simulink model "TB04_StageB_ClosedLoop"  (R2025a)
settings: Solver=FixedStepDiscrete  StartTime=0  StopTime=TB.t_end  FixedStep=TB.dt  RelTol=1e-3
InitFcn:
  | % 모델과 같은 폴더의 초기화 스크립트를 실행해 P(설계 파라미터)와 TB(시험 조건)를 만든다.
  | run(fullfile(fileparts(get_param(bdroot, 'FileName')), 'TB04_init.m'));
values from neighbouring files (symbols this model uses):
  TB = struct()    [TB04_init.m]
libraries: fl_lib x56, nesl_utility x23
(part 1 of 2)
settings Model: Creator=hj000  LastModifiedBy=hj000
settings DataIOCC: SaveOutput=off  SignalLogging=off  SaveTime=off

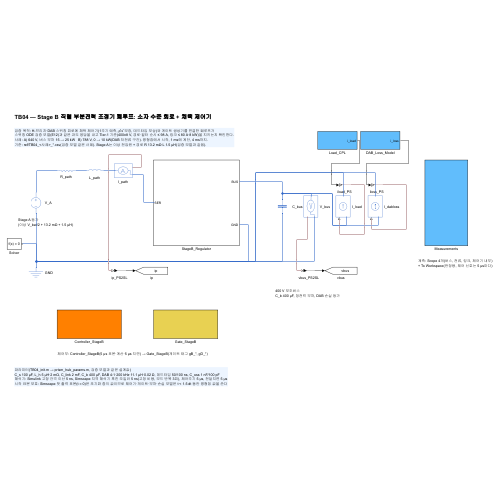
[thumbnail: Simulink's stored preview of the top-level diagram]
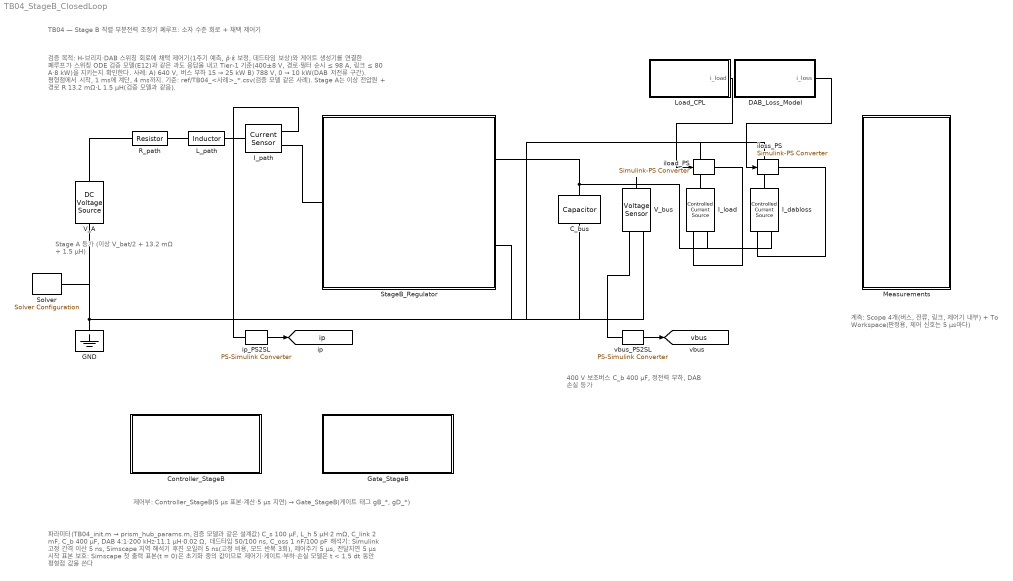
== system TB04_StageB_ClosedLoop ==
  note: TB04 — Stage B 직렬 부분전력 조정기 폐루프: 소자 수준 회로 + 채택 제어기
  note: 검증 목적: H-브리지·DAB 스위칭 회로에 채택 제어기(1주기 예측, ρ̂·ε̂ 보정, 데드타임 보상)와 게이트 생성기를 연결한 폐루프가
      | 스위칭 ODE 검증 모델(E12)과 같은 과도 응답을 내고 Tier-1 기준(400±8 V, 경로·필터 순시 ≤ 98 A, 링크 ≤ 80 A·8 kW)을 지키는지 확인한다.
      | 사례: A) 640 V, 버스 부하 15 → 25 kW   B) 788 V, 0 → 10 kW(DAB 저전류 구간). 평형점에서 시작, 1 ms에 계단, 4 ms까지.
      | 기준: ref/TB04_<사례>_*.csv(검증 모델 같은 사례). Stage A는 이상 전압원 + 경로 R 13.2 mΩ·L 1.5 µH(검증 모델과 같음).
  note: Stage A 등가
      | (이상 V_bat/2 + 13.2 mΩ + 1.5 µH)
  note: 400 V 보조버스
      | C_b 400 µF, 정전력 부하, DAB 손실 등가
  note: 제어부: Controller_StageB(5 µs 표본·계산·5 µs 지연) → Gate_StageB(게이트 태그 gB_*, gD_*)
  note: 계측: Scope 4개(버스, 전류, 링크, 제어기 내부)
      | + To Workspace(판정용, 제어 신호는 5 µs마다)
  note: 파라미터(TB04_init.m → prism_hub_params.m, 검증 모델과 같은 설계값)
      | C_s 100 µF, L_h 5 µH·2 mΩ, C_link 2 mF, C_b 400 µF, DAB 4:1·200 kHz·11.1 µH·0.02 Ω, 데드타임 50/100 ns, C_oss 1 nF/100 pF
      | 해석기: Simulink 고정 간격 이산 5 ns, Simscape 지역 해석기 후진 오일러 5 ns(고정 비용, 모드 반복 3회), 제어주기 5 µs, 전달지연 5 µs
      | 시작 표본 보호: Simscape 첫 출력 표본(t = 0)은 초기화 중의 값이므로 제어기·게이트·부하·손실 모델은 t < 1.5 dt 동안 평형점 값을 쓴다
  C_bus : fl_lib/Electrical/Electrical Elements/Capacitor  c=TB.Cb F  r=1e-6 Ohm  g=0 1/Ohm  i_specify=off  i_priority=None  i=0 A  i_nominal_specify=off  i_nominal_value=1  i_nominal_unit=A  v_specify=off  v_priority=None  v=0 V  v_nominal_specify=off  v_nominal_value=1  v_nominal_unit=V  vc_specify=on  vc_priority=High  vc=TB.vb0 V  vc_nominal_specify=off  vc_nominal_value=1  vc_nominal_unit=V
  Controller_StageB : Subsystem
  DAB_Loss_Model : Subsystem
  GND : fl_lib/Electrical/Electrical Elements/Electrical Reference
  Gate_StageB : Subsystem
  I_dabloss : fl_lib/Electrical/Electrical Sources/Controlled Current Source
  I_load : fl_lib/Electrical/Electrical Sources/Controlled Current Source
  I_path : fl_lib/Electrical/Electrical Sensors/Current Sensor
  L_path : fl_lib/Electrical/Electrical Elements/Inductor  l=TB.Lpath H  r=0 Ohm  g=1e-9 1/Ohm  i_specify=off  i_priority=None  i=0 A  i_nominal_specify=off  i_nominal_value=1  i_nominal_unit=A  v_specify=off  v_priority=None  v=0 V  v_nominal_specify=off  v_nominal_value=1  v_nominal_unit=V  i_L_specify=on  i_L_priority=High  i_L=TB.ip0 A  i_L_nominal_specify=off  i_L_nominal_value=1  i_L_nominal_unit=A
  Load_CPL : Subsystem
  Measurements : Subsystem
  R_path : fl_lib/Electrical/Electrical Elements/Resistor  R=TB.Rpath Ohm  i_specify=off  i_priority=None  i=0 A  i_nominal_specify=off  i_nominal_value=1  i_nominal_unit=A  v_specify=off  v_priority=None  v=0 V  v_nominal_specify=off  v_nominal_value=1  v_nominal_unit=V
  Solver : nesl_utility/Solver Configuration  PhysicalDomain=network_engine_domain  SubClassName=solver  LeftPortType=input  RightPortType=generic  Tones=[]  Harmonics=[]  SimulateNoise=off  Profile=off  UseLocalSampling=off  EnableSwitchedLinearOptims=on  FrequencyDomain=off  UseCCode=off  RelTol=0.001  AbsTol=0.001  MinStep=1e-09  ToWorkspace=off  RevertToSquareIcSolve=off  NumHomotopyIterations=100  PhasorMode=off  PhasorModeNumHarmonics=1  ConsistencySolver=NEWTON_XTOL_AFTER_FTOL  IndexReductionMethod=DerivativeReplacement  DoDC=off  ResidualTolerance=1e-9  ConsistencyTolSource=GLOBAL  ConsistencyAbsTol=0.001  ConsistencyRelTol=0.001  ConsistencyTolFactor=0.001  UseLocalSolver=on  LocalSolverChoice=NE_BACKWARD_EULER_ADVANCER  ResolveIndetEquations=on  FunctionEvalNumThread=1  LocalSolverSampleTime=TB.dt  DoFixedCost=on  MaxNonlinIter=3  MaxModeIter=2  ComputeImpulses=off  ImpulseIterations=2  LinearAlgebra=auto  LinearAlgebraNumThread=0  EquationFormulation=NE_TIME_EF  DelaysMemoryBudget=1024  AutomaticFiltering=on  FilteringTimeConstant=0.001  PartitionStorageMethod=AS_NEEDED  PartitionMemoryBudget=1024  PartitionMethod=ROBUST  MultibodyUseLocalSolver=off  MultibodyLocalSolverChoice=ODE1  MultibodyLocalSolverSampleTime=0.001
  StageB_Regulator : Subsystem
  V_A : fl_lib/Electrical/Electrical Sources/DC Voltage Source  v0=TB.VA V
  V_bus : fl_lib/Electrical/Electrical Sensors/Voltage Sensor
  iload_PS : nesl_utility/Simulink-PS Converter  PhysicalDomain=network_engine_domain  SubClassName=ps_input  LeftPortType=input  RightPortType=output  PseudoPeriodic=off  Frequencies=[]  NoiseDistribution=none  NoiseParameters=[]  Unit=1  AffineConversion=off  FilteringAndDerivatives=provide  SimscapeFilterOrder=1  InputFilterTimeConstant=0.001  UdotUserProvided=0
  iloss_PS : nesl_utility/Simulink-PS Converter  PhysicalDomain=network_engine_domain  SubClassName=ps_input  LeftPortType=input  RightPortType=output  PseudoPeriodic=off  Frequencies=[]  NoiseDistribution=none  NoiseParameters=[]  Unit=1  AffineConversion=off  FilteringAndDerivatives=provide  SimscapeFilterOrder=1  InputFilterTimeConstant=0.001  UdotUserProvided=0
  ip_PS2SL : nesl_utility/PS-Simulink Converter  PhysicalDomain=network_engine_domain  SubClassName=ps_output  LeftPortType=input  RightPortType=output  PseudoPeriodic=off  Frequencies=[]  VectorFormat=inherit  Unit=inherit  AffineConversion=off
  vbus_PS2SL : nesl_utility/PS-Simulink Converter  PhysicalDomain=network_engine_domain  SubClassName=ps_output  LeftPortType=input  RightPortType=output  PseudoPeriodic=off  Frequencies=[]  VectorFormat=inherit  Unit=inherit  AffineConversion=off
  tag scope: ip=global, vbus=global
  wires:
  ip_PS2SL/1 -> [ip]
  vbus_PS2SL/1 -> [vbus]
  Load_CPL/1(i_load) -> iload_PS/1
  DAB_Loss_Model/1(i_loss) -> iloss_PS/1
  connections:
  Solver/RConn1 -- V_A/RConn1 -- StageB_Regulator/RConn2 -- C_bus/RConn1 -- V_bus/RConn2 -- I_load/LConn1 -- GND/LConn1 -- I_dabloss/LConn1
  V_A/LConn1 -- R_path/LConn1
  R_path/RConn1 -- L_path/LConn1
  L_path/RConn1 -- I_path/LConn1
  I_path/RConn2 -- StageB_Regulator/LConn1
  StageB_Regulator/RConn1 -- V_bus/LConn1 -- I_load/RConn2 -- C_bus/LConn1 -- I_dabloss/RConn2
  iload_PS/RConn1 -- I_load/RConn1
  iloss_PS/RConn1 -- I_dabloss/RConn1
  I_path/RConn1 -- ip_PS2SL/LConn1
  V_bus/RConn1 -- vbus_PS2SL/LConn1

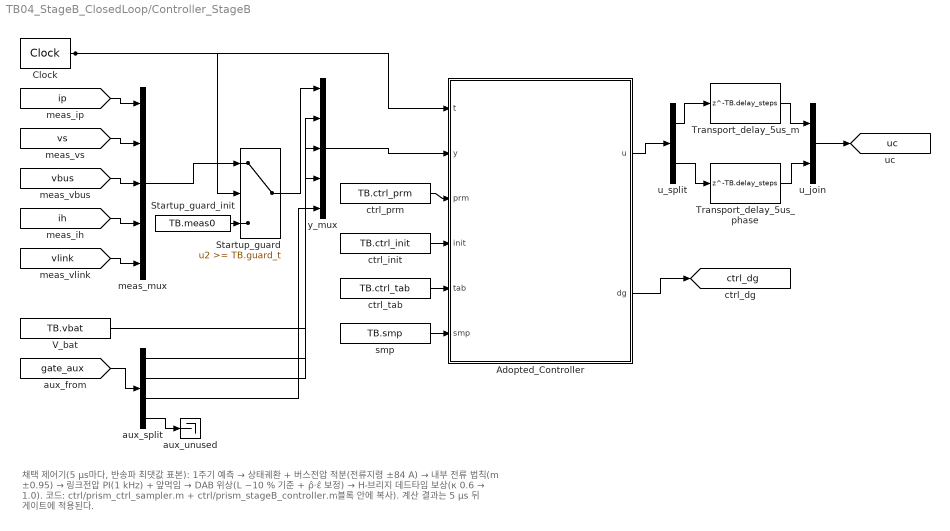
== system TB04_StageB_ClosedLoop/Controller_StageB ==
  note: 채택 제어기(5 µs마다, 반송파 최댓값 표본): 1주기 예측 → 상태궤환 + 버스전압 적분(전류지령 ±84 A) → 내부 전류 법칙(m ±0.95)
      | → 링크전압 PI(1 kHz) + 앞먹임 → DAB 위상(L −10 % 기준 + ρ̂·ε̂ 보정) → H-브리지 데드타임 보상(κ 0.6 → 1.0).
      | 코드: ctrl/prism_ctrl_sampler.m + ctrl/prism_stageB_controller.m(블록 안에 복사). 계산 결과는 5 µs 뒤 게이트에 적용된다.
  Adopted_Controller : MATLAB Function  TreatAsAtomicUnit=on
  Clock : DigitalClock  SampleTime=TB.dt
  Startup_guard : Switch  Threshold=TB.guard_t  SaturateOnIntegerOverflow=off  InputSameDT=off
  Startup_guard_init : Constant  Value=TB.meas0
  Transport_delay_5us_m : Delay  DelayLength=TB.delay_steps  InitialCondition=TB.uc0(1)
  Transport_delay_5us_phase : Delay  DelayLength=TB.delay_steps  InitialCondition=TB.uc0(2)
  V_bat : Constant  Value=TB.vbat
  aux_split : Demux  Outputs=[1 1 1 3]
  aux_unused : Terminator
  ctrl_init : Constant  Value=TB.ctrl_init
  ctrl_prm : Constant  Value=TB.ctrl_prm
  ctrl_tab : Constant  Value=TB.ctrl_tab
  meas_mux : Mux  Inputs=5
  smp : Constant  Value=TB.smp
  u_join : Mux  Inputs=2
  u_split : Demux  Outputs=2
  y_mux : Mux  Inputs=5
  tag scope: ctrl_dg=global, uc=global
  wires:
  [ip] -> meas_mux/1
  [vs] -> meas_mux/2
  [vbus] -> meas_mux/3
  [ih] -> meas_mux/4
  [vlink] -> meas_mux/5
  Startup_guard_init/1 -> Startup_guard/3
  meas_mux/1 -> Startup_guard/1
  Clock/1 -> Startup_guard/2, Adopted_Controller/1(t)
  Startup_guard/1 -> y_mux/1
  V_bat/1 -> y_mux/2
  [gate_aux] -> aux_split/1
  aux_split/1 -> y_mux/3
  aux_split/2 -> y_mux/4
  aux_split/3 -> y_mux/5
  aux_split/4 -> aux_unused/1
  y_mux/1 -> Adopted_Controller/2(y)
  ctrl_prm/1 -> Adopted_Controller/3(prm)
  ctrl_init/1 -> Adopted_Controller/4(init)
  ctrl_tab/1 -> Adopted_Controller/5(tab)
  smp/1 -> Adopted_Controller/6(smp)
  Adopted_Controller/1(u) -> u_split/1
  u_split/1 -> Transport_delay_5us_m/1
  u_split/2 -> Transport_delay_5us_phase/1
  Transport_delay_5us_m/1 -> u_join/1
  Transport_delay_5us_phase/1 -> u_join/2
  u_join/1 -> [uc]
  Adopted_Controller/2(dg) -> [ctrl_dg]

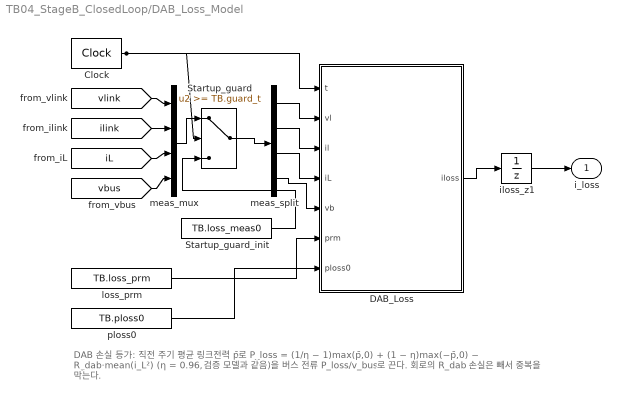
== system TB04_StageB_ClosedLoop/DAB_Loss_Model ==
  note: DAB 손실 등가: 직전 주기 평균 링크전력 p̄로 P_loss = (1/η − 1)max(p̄,0) + (1 − η)max(−p̄,0) − R_dab·mean(i_L²)
      | (η = 0.96, 검증 모델과 같음)을 버스 전류 P_loss/v_bus로 끈다. 회로의 R_dab 손실은 빼서 중복을 막는다.
  Clock : DigitalClock  SampleTime=TB.dt
  DAB_Loss : MATLAB Function  TreatAsAtomicUnit=on
  Startup_guard : Switch  Threshold=TB.guard_t  SaturateOnIntegerOverflow=off  InputSameDT=off
  Startup_guard_init : Constant  Value=TB.loss_meas0
  iloss_z1 : UnitDelay  SampleTime=TB.dt  HasFrameUpgradeWarning=on
  loss_prm : Constant  Value=TB.loss_prm
  meas_mux : Mux
  meas_split : Demux
  ploss0 : Constant  Value=TB.ploss0
  i_loss : Outport
  wires:
  [vlink] -> meas_mux/1
  [ilink] -> meas_mux/2
  [iL] -> meas_mux/3
  [vbus] -> meas_mux/4
  Startup_guard_init/1 -> Startup_guard/3
  meas_mux/1 -> Startup_guard/1
  Clock/1 -> Startup_guard/2, DAB_Loss/1(t)
  Startup_guard/1 -> meas_split/1
  meas_split/1 -> DAB_Loss/2(vl)
  meas_split/2 -> DAB_Loss/3(il)
  meas_split/3 -> DAB_Loss/4(iL)
  meas_split/4 -> DAB_Loss/5(vb)
  loss_prm/1 -> DAB_Loss/6(prm)
  ploss0/1 -> DAB_Loss/7(ploss0)
  DAB_Loss/1(iloss) -> iloss_z1/1
  iloss_z1/1 -> i_loss/1

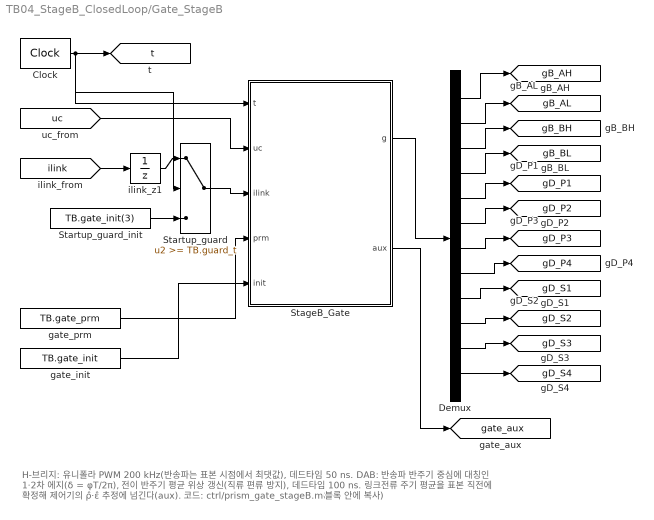
== system TB04_StageB_ClosedLoop/Gate_StageB ==
  note: H-브리지: 유니폴라 PWM 200 kHz(반송파는 표본 시점에서 최댓값), 데드타임 50 ns.
      | DAB: 반송파 반주기 중심에 대칭인 1·2차 에지(δ = φT/2π), 전이 반주기 평균 위상 갱신(직류 편류 방지), 데드타임 100 ns.
      | 링크전류 주기 평균을 표본 직전에 확정해 제어기의 ρ̂·ε̂ 추정에 넘긴다(aux). 코드: ctrl/prism_gate_stageB.m(블록 안에 복사)
  Clock : DigitalClock  SampleTime=TB.dt
  Demux : Demux  Outputs=12
  StageB_Gate : MATLAB Function  TreatAsAtomicUnit=on
  Startup_guard : Switch  Threshold=TB.guard_t  SaturateOnIntegerOverflow=off  InputSameDT=off
  Startup_guard_init : Constant  Value=TB.gate_init(3)
  gate_init : Constant  Value=TB.gate_init
  gate_prm : Constant  Value=TB.gate_prm
  ilink_z1 : UnitDelay  SampleTime=TB.dt  HasFrameUpgradeWarning=on
  tag scope: gB_AH=global, gB_AL=global, gB_BH=global, gB_BL=global, gD_P1=global, gD_P2=global, gD_P3=global, gD_P4=global, gD_S1=global, gD_S2=global, gD_S3=global, gD_S4=global, gate_aux=global, t=global
  wires:
  Startup_guard_init/1 -> Startup_guard/3
  Clock/1 -> [t], StageB_Gate/1(t), Startup_guard/2
  [uc] -> StageB_Gate/2(uc)
  [ilink] -> ilink_z1/1
  ilink_z1/1 -> Startup_guard/1
  Startup_guard/1 -> StageB_Gate/3(ilink)
  gate_prm/1 -> StageB_Gate/4(prm)
  gate_init/1 -> StageB_Gate/5(init)
  StageB_Gate/1(g) -> Demux/1
  Demux/1 -> [gB_AH]
  Demux/2 -> [gB_AL]
  Demux/3 -> [gB_BH]
  Demux/4 -> [gB_BL]
  Demux/5 -> [gD_P1]
  Demux/6 -> [gD_P2]
  Demux/7 -> [gD_P3]
  Demux/8 -> [gD_P4]
  Demux/9 -> [gD_S1]
  Demux/10 -> [gD_S2]
  Demux/11 -> [gD_S3]
  Demux/12 -> [gD_S4]
  StageB_Gate/2(aux) -> [gate_aux]

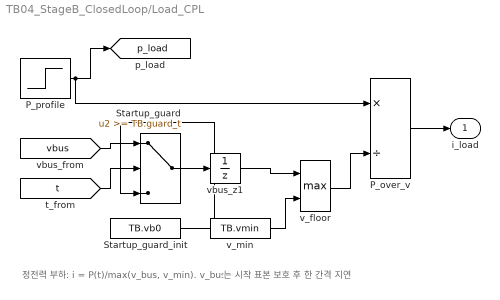
== system TB04_StageB_ClosedLoop/Load_CPL ==
  note: 정전력 부하: i = P(t)/max(v_bus, v_min). v_bus는 시작 표본 보호 후 한 간격 지연
  P_over_v : Product  Inputs=*/
  P_profile : Step  Time=TB.t_step  Before=TB.P0  After=TB.P1  SampleTime=TB.dt
  Startup_guard : Switch  Threshold=TB.guard_t  SaturateOnIntegerOverflow=off  InputSameDT=off
  Startup_guard_init : Constant  Value=TB.vb0
  v_floor : MinMax  Function=max  Inputs=2
  v_min : Constant  Value=TB.vmin
  vbus_z1 : UnitDelay  SampleTime=TB.dt  HasFrameUpgradeWarning=on
  i_load : Outport
  tag scope: p_load=global
  wires:
  Startup_guard_init/1 -> Startup_guard/3
  P_profile/1 -> [p_load], P_over_v/1
  [vbus] -> Startup_guard/1
  [t] -> Startup_guard/2
  Startup_guard/1 -> vbus_z1/1
  vbus_z1/1 -> v_floor/1
  v_min/1 -> v_floor/2
  v_floor/1 -> P_over_v/2
  P_over_v/1 -> i_load/1

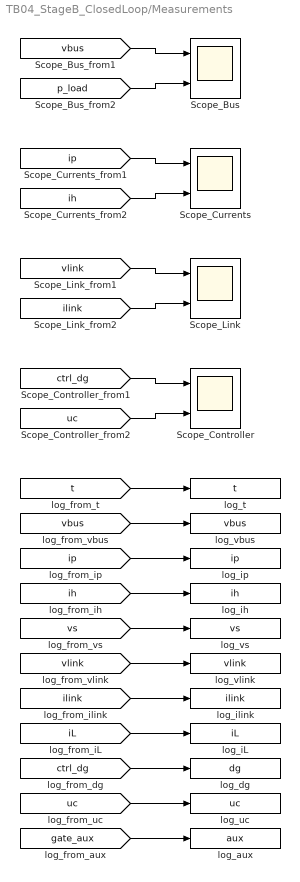
== system TB04_StageB_ClosedLoop/Measurements ==
  Scope_Bus : Scope  NumInputPorts=2
      settings: Title=Scope Bus
  Scope_Controller : Scope  NumInputPorts=2
      settings: Title=Scope Controller
  Scope_Currents : Scope  NumInputPorts=2
      settings: Title=Scope Currents
  Scope_Link : Scope  NumInputPorts=2
      settings: Title=Scope Link
  log_aux : ToWorkspace  VariableName=aux  SampleTime=-1
      settings: Decimation=TB.Np
  log_dg : ToWorkspace  VariableName=dg  SampleTime=-1
      settings: Decimation=TB.Np
  log_iL : ToWorkspace  VariableName=iL  SampleTime=-1
  log_ih : ToWorkspace  VariableName=ih  SampleTime=-1
  log_ilink : ToWorkspace  VariableName=ilink  SampleTime=-1
  log_ip : ToWorkspace  VariableName=ip  SampleTime=-1
  log_t : ToWorkspace  VariableName=t  SampleTime=-1
  log_uc : ToWorkspace  VariableName=uc  SampleTime=-1
      settings: Decimation=TB.Np
  log_vbus : ToWorkspace  VariableName=vbus  SampleTime=-1
  log_vlink : ToWorkspace  VariableName=vlink  SampleTime=-1
  log_vs : ToWorkspace  VariableName=vs  SampleTime=-1
  wires:
  [vbus] -> Scope_Bus/1
  [p_load] -> Scope_Bus/2
  [ip] -> Scope_Currents/1
  [ih] -> Scope_Currents/2
  [vlink] -> Scope_Link/1
  [ilink] -> Scope_Link/2
  [ctrl_dg] -> Scope_Controller/1
  [uc] -> Scope_Controller/2
  [t] -> log_t/1
  [vbus] -> log_vbus/1
  [ip] -> log_ip/1
  [ih] -> log_ih/1
  [vs] -> log_vs/1
  [vlink] -> log_vlink/1
  [ilink] -> log_ilink/1
  [iL] -> log_iL/1
  [ctrl_dg] -> log_dg/1
  [uc] -> log_uc/1
  [gate_aux] -> log_aux/1

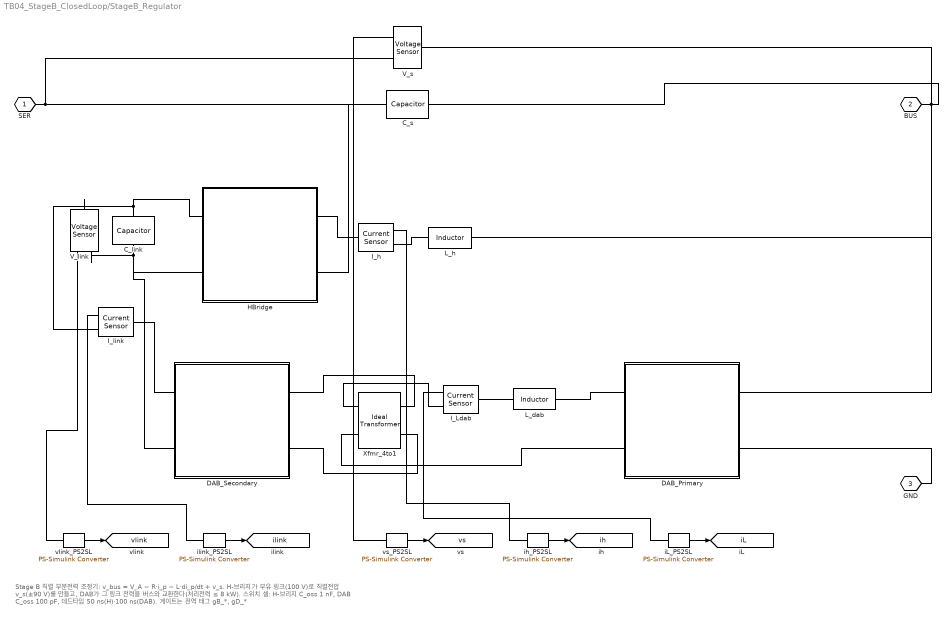
== system TB04_StageB_ClosedLoop/StageB_Regulator ==
  note: Stage B 직렬 부분전력 조정기: v_bus = V_A − R·i_p − L·di_p/dt + v_s.
      | H-브리지가 부유 링크(100 V)로 직렬전압 v_s(±90 V)를 만들고, DAB가 그 링크 전력을 버스와 교환한다(처리전력 ≤ 8 kW).
      | 스위치 셀: H-브리지 C_oss 1 nF, DAB C_oss 100 pF, 데드타임 50 ns(H)·100 ns(DAB). 게이트는 전역 태그 gB_*, gD_*
  C_link : fl_lib/Electrical/Electrical Elements/Capacitor  c=TB.B.Clink F  r=1e-6 Ohm  g=0 1/Ohm  i_specify=off  i_priority=None  i=0 A  i_nominal_specify=off  i_nominal_value=1  i_nominal_unit=A  v_specify=off  v_priority=None  v=0 V  v_nominal_specify=off  v_nominal_value=1  v_nominal_unit=V  vc_specify=on  vc_priority=High  vc=TB.vl0 V  vc_nominal_specify=off  vc_nominal_value=1  vc_nominal_unit=V
  C_s : fl_lib/Electrical/Electrical Elements/Capacitor  c=TB.B.Cs F  r=1e-6 Ohm  g=0 1/Ohm  i_specify=off  i_priority=None  i=0 A  i_nominal_specify=off  i_nominal_value=1  i_nominal_unit=A  v_specify=off  v_priority=None  v=0 V  v_nominal_specify=off  v_nominal_value=1  v_nominal_unit=V  vc_specify=on  vc_priority=High  vc=TB.vs0 V  vc_nominal_specify=off  vc_nominal_value=1  vc_nominal_unit=V
  DAB_Primary : Subsystem
  DAB_Secondary : Subsystem
  HBridge : Subsystem
  I_Ldab : fl_lib/Electrical/Electrical Sensors/Current Sensor
  I_h : fl_lib/Electrical/Electrical Sensors/Current Sensor
  I_link : fl_lib/Electrical/Electrical Sensors/Current Sensor
  L_dab : fl_lib/Electrical/Electrical Elements/Inductor  l=TB.B.Ldab H  r=TB.B.Rdab Ohm  g=1e-9 1/Ohm  i_specify=off  i_priority=None  i=0 A  i_nominal_specify=off  i_nominal_value=1  i_nominal_unit=A  v_specify=off  v_priority=None  v=0 V  v_nominal_specify=off  v_nominal_value=1  v_nominal_unit=V  i_L_specify=on  i_L_priority=High  i_L=0 A  i_L_nominal_specify=off  i_L_nominal_value=1  i_L_nominal_unit=A
  L_h : fl_lib/Electrical/Electrical Elements/Inductor  l=TB.B.Lh H  r=TB.B.Rh Ohm  g=1e-9 1/Ohm  i_specify=off  i_priority=None  i=0 A  i_nominal_specify=off  i_nominal_value=1  i_nominal_unit=A  v_specify=off  v_priority=None  v=0 V  v_nominal_specify=off  v_nominal_value=1  v_nominal_unit=V  i_L_specify=on  i_L_priority=High  i_L=TB.ih0 A  i_L_nominal_specify=off  i_L_nominal_value=1  i_L_nominal_unit=A
  V_link : fl_lib/Electrical/Electrical Sensors/Voltage Sensor
  V_s : fl_lib/Electrical/Electrical Sensors/Voltage Sensor
  Xfmr_4to1 : fl_lib/Electrical/Electrical Elements/Ideal Transformer  n=TB.B.n  i1_specify=off  i1_priority=None  i1=0 A  i1_nominal_specify=off  i1_nominal_value=1  i1_nominal_unit=A  v1_specify=off  v1_priority=None  v1=0 V  v1_nominal_specify=off  v1_nominal_value=1  v1_nominal_unit=V  i2_specify=off  i2_priority=None  i2=0 A  i2_nominal_specify=off  i2_nominal_value=1  i2_nominal_unit=A  v2_specify=off  v2_priority=None  v2=0 V  v2_nominal_specify=off  v2_nominal_value=1  v2_nominal_unit=V
  iL_PS2SL : nesl_utility/PS-Simulink Converter  PhysicalDomain=network_engine_domain  SubClassName=ps_output  LeftPortType=input  RightPortType=output  PseudoPeriodic=off  Frequencies=[]  VectorFormat=inherit  Unit=inherit  AffineConversion=off
  ih_PS2SL : nesl_utility/PS-Simulink Converter  PhysicalDomain=network_engine_domain  SubClassName=ps_output  LeftPortType=input  RightPortType=output  PseudoPeriodic=off  Frequencies=[]  VectorFormat=inherit  Unit=inherit  AffineConversion=off
  ilink_PS2SL : nesl_utility/PS-Simulink Converter  PhysicalDomain=network_engine_domain  SubClassName=ps_output  LeftPortType=input  RightPortType=output  PseudoPeriodic=off  Frequencies=[]  VectorFormat=inherit  Unit=inherit  AffineConversion=off
  vlink_PS2SL : nesl_utility/PS-Simulink Converter  PhysicalDomain=network_engine_domain  SubClassName=ps_output  LeftPortType=input  RightPortType=output  PseudoPeriodic=off  Frequencies=[]  VectorFormat=inherit  Unit=inherit  AffineConversion=off
  vs_PS2SL : nesl_utility/PS-Simulink Converter  PhysicalDomain=network_engine_domain  SubClassName=ps_output  LeftPortType=input  RightPortType=output  PseudoPeriodic=off  Frequencies=[]  VectorFormat=inherit  Unit=inherit  AffineConversion=off
  SER : PMIOPort  Side=Left
  BUS : PMIOPort  Port=2  Side=Right
  GND : PMIOPort  Port=3  Side=Right
  tag scope: iL=global, ih=global, ilink=global, vlink=global, vs=global
  wires:
  vs_PS2SL/1 -> [vs]
  ih_PS2SL/1 -> [ih]
  vlink_PS2SL/1 -> [vlink]
  ilink_PS2SL/1 -> [ilink]
  iL_PS2SL/1 -> [iL]
  connections:
  C_s/RConn1 -- V_s/RConn2 -- SER/RConn1 -- HBridge/RConn2
  C_s/LConn1 -- V_s/LConn1 -- L_h/RConn1 -- BUS/RConn1 -- DAB_Primary/LConn1
  HBridge/RConn1 -- I_h/LConn1
  I_h/RConn2 -- L_h/LConn1
  HBridge/LConn1 -- C_link/LConn1 -- V_link/LConn1 -- I_link/RConn2
  HBridge/LConn2 -- C_link/RConn1 -- V_link/RConn2 -- DAB_Secondary/LConn2
  DAB_Secondary/LConn1 -- I_link/LConn1
  DAB_Secondary/RConn1 -- Xfmr_4to1/RConn1
  DAB_Secondary/RConn2 -- Xfmr_4to1/RConn2
  DAB_Primary/RConn1 -- L_dab/LConn1
  L_dab/RConn1 -- I_Ldab/LConn1
  I_Ldab/RConn2 -- Xfmr_4to1/LConn1
  Xfmr_4to1/LConn2 -- DAB_Primary/RConn2
  DAB_Primary/LConn2 -- GND/RConn1
  V_s/RConn1 -- vs_PS2SL/LConn1
  I_h/RConn1 -- ih_PS2SL/LConn1
  V_link/RConn1 -- vlink_PS2SL/LConn1
  I_link/RConn1 -- ilink_PS2SL/LConn1
  I_Ldab/RConn1 -- iL_PS2SL/LConn1

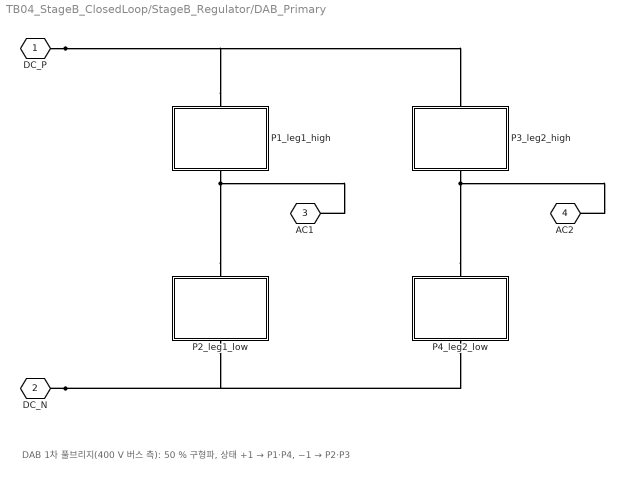
== system TB04_StageB_ClosedLoop/StageB_Regulator/DAB_Primary ==
  note: DAB 1차 풀브리지(400 V 버스 측): 50 % 구형파, 상태 +1 → P1·P4, −1 → P2·P3
  P1_leg1_high : Subsystem  mask(PRISM-Hub switch cell){Ron=TB.B.Ron, Goff=TB.B.Goff, Vf=TB.B.Vf, Rd=TB.B.Rd, Goffd=TB.B.Goffd, Coss=TB.B.Coss_d}
      mask prompts: Ron "도통 저항 R_on [Ohm]"; Goff "차단 컨덕턴스 G_off [S]"; Vf "다이오드 순방향 전압 Vf [V]"; Rd "다이오드 도통 저항 R_d [Ohm]"; Goffd "다이오드 차단 컨덕턴스 [S]"; Coss "출력용량 C_oss [F]"
      mask help: 전력 반도체 스위치 셀 P1_leg1_high. 게이트 태그 gD_P1.
      settings: AttributesFormatString=gate: gD_P1
      mask Display:
      | plot([0.50 0.50 ],[0.95 0.65 ],[0.50 0.74 ],[0.65 0.35 ],[0.50 0.50 ],[0.35 0.05 ]);
      | plot([0.50 0.20 0.20 ],[0.80 0.80 0.58 ],[0.20 0.20 0.50 ],[0.42 0.20 0.20 ]);
      | plot([0.20 0.10 0.30 0.20 ],[0.58 0.42 0.42 0.58 ],[0.10 0.30 ],[0.58 0.58 ]);
      | port_label('LConn',1,'D');
      | port_label('RConn',1,'S');
  P2_leg1_low : Subsystem  mask(PRISM-Hub switch cell){Ron=TB.B.Ron, Goff=TB.B.Goff, Vf=TB.B.Vf, Rd=TB.B.Rd, Goffd=TB.B.Goffd, Coss=TB.B.Coss_d}
      mask prompts: Ron "도통 저항 R_on [Ohm]"; Goff "차단 컨덕턴스 G_off [S]"; Vf "다이오드 순방향 전압 Vf [V]"; Rd "다이오드 도통 저항 R_d [Ohm]"; Goffd "다이오드 차단 컨덕턴스 [S]"; Coss "출력용량 C_oss [F]"
      mask help: 전력 반도체 스위치 셀 P2_leg1_low. 게이트 태그 gD_P2.
      settings: AttributesFormatString=gate: gD_P2
      mask Display:
      | plot([0.50 0.50 ],[0.95 0.65 ],[0.50 0.74 ],[0.65 0.35 ],[0.50 0.50 ],[0.35 0.05 ]);
      | plot([0.50 0.20 0.20 ],[0.80 0.80 0.58 ],[0.20 0.20 0.50 ],[0.42 0.20 0.20 ]);
      | plot([0.20 0.10 0.30 0.20 ],[0.58 0.42 0.42 0.58 ],[0.10 0.30 ],[0.58 0.58 ]);
      | port_label('LConn',1,'D');
      | port_label('RConn',1,'S');
  P3_leg2_high : Subsystem  mask(PRISM-Hub switch cell){Ron=TB.B.Ron, Goff=TB.B.Goff, Vf=TB.B.Vf, Rd=TB.B.Rd, Goffd=TB.B.Goffd, Coss=TB.B.Coss_d}
      mask prompts: Ron "도통 저항 R_on [Ohm]"; Goff "차단 컨덕턴스 G_off [S]"; Vf "다이오드 순방향 전압 Vf [V]"; Rd "다이오드 도통 저항 R_d [Ohm]"; Goffd "다이오드 차단 컨덕턴스 [S]"; Coss "출력용량 C_oss [F]"
      mask help: 전력 반도체 스위치 셀 P3_leg2_high. 게이트 태그 gD_P3.
      settings: AttributesFormatString=gate: gD_P3
      mask Display:
      | plot([0.50 0.50 ],[0.95 0.65 ],[0.50 0.74 ],[0.65 0.35 ],[0.50 0.50 ],[0.35 0.05 ]);
      | plot([0.50 0.20 0.20 ],[0.80 0.80 0.58 ],[0.20 0.20 0.50 ],[0.42 0.20 0.20 ]);
      | plot([0.20 0.10 0.30 0.20 ],[0.58 0.42 0.42 0.58 ],[0.10 0.30 ],[0.58 0.58 ]);
      | port_label('LConn',1,'D');
      | port_label('RConn',1,'S');
  P4_leg2_low : Subsystem  mask(PRISM-Hub switch cell){Ron=TB.B.Ron, Goff=TB.B.Goff, Vf=TB.B.Vf, Rd=TB.B.Rd, Goffd=TB.B.Goffd, Coss=TB.B.Coss_d}
      mask prompts: Ron "도통 저항 R_on [Ohm]"; Goff "차단 컨덕턴스 G_off [S]"; Vf "다이오드 순방향 전압 Vf [V]"; Rd "다이오드 도통 저항 R_d [Ohm]"; Goffd "다이오드 차단 컨덕턴스 [S]"; Coss "출력용량 C_oss [F]"
      mask help: 전력 반도체 스위치 셀 P4_leg2_low. 게이트 태그 gD_P4.
      settings: AttributesFormatString=gate: gD_P4
      mask Display:
      | plot([0.50 0.50 ],[0.95 0.65 ],[0.50 0.74 ],[0.65 0.35 ],[0.50 0.50 ],[0.35 0.05 ]);
      | plot([0.50 0.20 0.20 ],[0.80 0.80 0.58 ],[0.20 0.20 0.50 ],[0.42 0.20 0.20 ]);
      | plot([0.20 0.10 0.30 0.20 ],[0.58 0.42 0.42 0.58 ],[0.10 0.30 ],[0.58 0.58 ]);
      | port_label('LConn',1,'D');
      | port_label('RConn',1,'S');
  DC_P : PMIOPort  Side=Left
  DC_N : PMIOPort  Port=2  Side=Left
  AC1 : PMIOPort  Port=3  Side=Right
  AC2 : PMIOPort  Port=4  Side=Right
  connections:
  P1_leg1_high/LConn1 -- DC_P/RConn1 -- P3_leg2_high/LConn1
  P2_leg1_low/LConn1 -- P1_leg1_high/RConn1 -- AC1/RConn1
  P4_leg2_low/LConn1 -- P3_leg2_high/RConn1 -- AC2/RConn1
  DC_N/RConn1 -- P2_leg1_low/RConn1 -- P4_leg2_low/RConn1

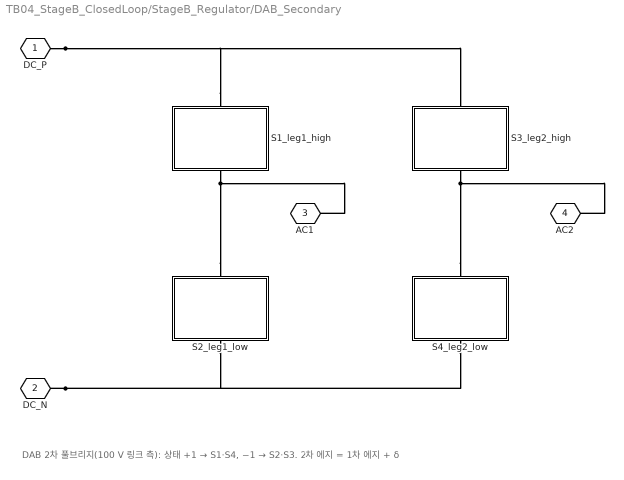
== system TB04_StageB_ClosedLoop/StageB_Regulator/DAB_Secondary ==
  note: DAB 2차 풀브리지(100 V 링크 측): 상태 +1 → S1·S4, −1 → S2·S3. 2차 에지 = 1차 에지 + δ
  S1_leg1_high : Subsystem  mask(PRISM-Hub switch cell){Ron=TB.B.Ron, Goff=TB.B.Goff, Vf=TB.B.Vf, Rd=TB.B.Rd, Goffd=TB.B.Goffd, Coss=TB.B.Coss_d}
      mask prompts: Ron "도통 저항 R_on [Ohm]"; Goff "차단 컨덕턴스 G_off [S]"; Vf "다이오드 순방향 전압 Vf [V]"; Rd "다이오드 도통 저항 R_d [Ohm]"; Goffd "다이오드 차단 컨덕턴스 [S]"; Coss "출력용량 C_oss [F]"
      mask help: 전력 반도체 스위치 셀 S1_leg1_high. 게이트 태그 gD_S1.
      settings: AttributesFormatString=gate: gD_S1
      mask Display:
      | plot([0.50 0.50 ],[0.95 0.65 ],[0.50 0.74 ],[0.65 0.35 ],[0.50 0.50 ],[0.35 0.05 ]);
      | plot([0.50 0.20 0.20 ],[0.80 0.80 0.58 ],[0.20 0.20 0.50 ],[0.42 0.20 0.20 ]);
      | plot([0.20 0.10 0.30 0.20 ],[0.58 0.42 0.42 0.58 ],[0.10 0.30 ],[0.58 0.58 ]);
      | port_label('LConn',1,'D');
      | port_label('RConn',1,'S');
  S2_leg1_low : Subsystem  mask(PRISM-Hub switch cell){Ron=TB.B.Ron, Goff=TB.B.Goff, Vf=TB.B.Vf, Rd=TB.B.Rd, Goffd=TB.B.Goffd, Coss=TB.B.Coss_d}
      mask prompts: Ron "도통 저항 R_on [Ohm]"; Goff "차단 컨덕턴스 G_off [S]"; Vf "다이오드 순방향 전압 Vf [V]"; Rd "다이오드 도통 저항 R_d [Ohm]"; Goffd "다이오드 차단 컨덕턴스 [S]"; Coss "출력용량 C_oss [F]"
      mask help: 전력 반도체 스위치 셀 S2_leg1_low. 게이트 태그 gD_S2.
      settings: AttributesFormatString=gate: gD_S2
      mask Display:
      | plot([0.50 0.50 ],[0.95 0.65 ],[0.50 0.74 ],[0.65 0.35 ],[0.50 0.50 ],[0.35 0.05 ]);
      | plot([0.50 0.20 0.20 ],[0.80 0.80 0.58 ],[0.20 0.20 0.50 ],[0.42 0.20 0.20 ]);
      | plot([0.20 0.10 0.30 0.20 ],[0.58 0.42 0.42 0.58 ],[0.10 0.30 ],[0.58 0.58 ]);
      | port_label('LConn',1,'D');
      | port_label('RConn',1,'S');
  S3_leg2_high : Subsystem  mask(PRISM-Hub switch cell){Ron=TB.B.Ron, Goff=TB.B.Goff, Vf=TB.B.Vf, Rd=TB.B.Rd, Goffd=TB.B.Goffd, Coss=TB.B.Coss_d}
      mask prompts: Ron "도통 저항 R_on [Ohm]"; Goff "차단 컨덕턴스 G_off [S]"; Vf "다이오드 순방향 전압 Vf [V]"; Rd "다이오드 도통 저항 R_d [Ohm]"; Goffd "다이오드 차단 컨덕턴스 [S]"; Coss "출력용량 C_oss [F]"
      mask help: 전력 반도체 스위치 셀 S3_leg2_high. 게이트 태그 gD_S3.
      settings: AttributesFormatString=gate: gD_S3
      mask Display:
      | plot([0.50 0.50 ],[0.95 0.65 ],[0.50 0.74 ],[0.65 0.35 ],[0.50 0.50 ],[0.35 0.05 ]);
      | plot([0.50 0.20 0.20 ],[0.80 0.80 0.58 ],[0.20 0.20 0.50 ],[0.42 0.20 0.20 ]);
      | plot([0.20 0.10 0.30 0.20 ],[0.58 0.42 0.42 0.58 ],[0.10 0.30 ],[0.58 0.58 ]);
      | port_label('LConn',1,'D');
      | port_label('RConn',1,'S');
  S4_leg2_low : Subsystem  mask(PRISM-Hub switch cell){Ron=TB.B.Ron, Goff=TB.B.Goff, Vf=TB.B.Vf, Rd=TB.B.Rd, Goffd=TB.B.Goffd, Coss=TB.B.Coss_d}
      mask prompts: Ron "도통 저항 R_on [Ohm]"; Goff "차단 컨덕턴스 G_off [S]"; Vf "다이오드 순방향 전압 Vf [V]"; Rd "다이오드 도통 저항 R_d [Ohm]"; Goffd "다이오드 차단 컨덕턴스 [S]"; Coss "출력용량 C_oss [F]"
      mask help: 전력 반도체 스위치 셀 S4_leg2_low. 게이트 태그 gD_S4.
      settings: AttributesFormatString=gate: gD_S4
      mask Display:
      | plot([0.50 0.50 ],[0.95 0.65 ],[0.50 0.74 ],[0.65 0.35 ],[0.50 0.50 ],[0.35 0.05 ]);
      | plot([0.50 0.20 0.20 ],[0.80 0.80 0.58 ],[0.20 0.20 0.50 ],[0.42 0.20 0.20 ]);
      | plot([0.20 0.10 0.30 0.20 ],[0.58 0.42 0.42 0.58 ],[0.10 0.30 ],[0.58 0.58 ]);
      | port_label('LConn',1,'D');
      | port_label('RConn',1,'S');
  DC_P : PMIOPort  Side=Left
  DC_N : PMIOPort  Port=2  Side=Left
  AC1 : PMIOPort  Port=3  Side=Right
  AC2 : PMIOPort  Port=4  Side=Right
  connections:
  S1_leg1_high/LConn1 -- DC_P/RConn1 -- S3_leg2_high/LConn1
  S2_leg1_low/LConn1 -- S1_leg1_high/RConn1 -- AC1/RConn1
  S4_leg2_low/LConn1 -- S3_leg2_high/RConn1 -- AC2/RConn1
  DC_N/RConn1 -- S2_leg1_low/RConn1 -- S4_leg2_low/RConn1

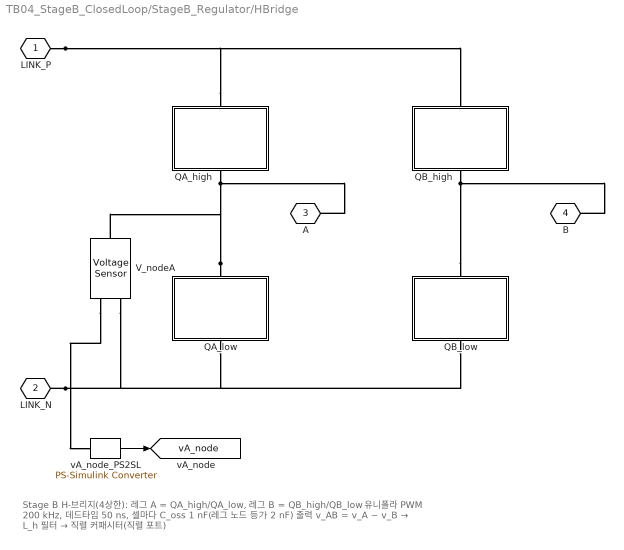
== system TB04_StageB_ClosedLoop/StageB_Regulator/HBridge ==
  note: Stage B H-브리지(4상한): 레그 A = QA_high/QA_low, 레그 B = QB_high/QB_low
      | 유니폴라 PWM 200 kHz, 데드타임 50 ns, 셀마다 C_oss 1 nF(레그 노드 등가 2 nF)
      | 출력 v_AB = v_A − v_B → L_h 필터 → 직렬 커패시터(직렬 포트)
  QA_high : Subsystem  mask(PRISM-Hub switch cell){Ron=TB.B.Ron, Goff=TB.B.Goff, Vf=TB.B.Vf, Rd=TB.B.Rd, Goffd=TB.B.Goffd, Coss=TB.B.Coss_h}
      mask prompts: Ron "도통 저항 R_on [Ohm]"; Goff "차단 컨덕턴스 G_off [S]"; Vf "다이오드 순방향 전압 Vf [V]"; Rd "다이오드 도통 저항 R_d [Ohm]"; Goffd "다이오드 차단 컨덕턴스 [S]"; Coss "출력용량 C_oss [F]"
      mask help: 전력 반도체 스위치 셀 QA_H. 게이트 태그 gB_AH.
      settings: AttributesFormatString=gate: gB_AH
      mask Display:
      | plot([0.50 0.50 ],[0.95 0.65 ],[0.50 0.74 ],[0.65 0.35 ],[0.50 0.50 ],[0.35 0.05 ]);
      | plot([0.50 0.20 0.20 ],[0.80 0.80 0.58 ],[0.20 0.20 0.50 ],[0.42 0.20 0.20 ]);
      | plot([0.20 0.10 0.30 0.20 ],[0.58 0.42 0.42 0.58 ],[0.10 0.30 ],[0.58 0.58 ]);
      | port_label('LConn',1,'D');
      | port_label('RConn',1,'S');
  QA_low : Subsystem  mask(PRISM-Hub switch cell){Ron=TB.B.Ron, Goff=TB.B.Goff, Vf=TB.B.Vf, Rd=TB.B.Rd, Goffd=TB.B.Goffd, Coss=TB.B.Coss_h}
      mask prompts: Ron "도통 저항 R_on [Ohm]"; Goff "차단 컨덕턴스 G_off [S]"; Vf "다이오드 순방향 전압 Vf [V]"; Rd "다이오드 도통 저항 R_d [Ohm]"; Goffd "다이오드 차단 컨덕턴스 [S]"; Coss "출력용량 C_oss [F]"
      mask help: 전력 반도체 스위치 셀 QA_L. 게이트 태그 gB_AL.
      settings: AttributesFormatString=gate: gB_AL
      mask Display:
      | plot([0.50 0.50 ],[0.95 0.65 ],[0.50 0.74 ],[0.65 0.35 ],[0.50 0.50 ],[0.35 0.05 ]);
      | plot([0.50 0.20 0.20 ],[0.80 0.80 0.58 ],[0.20 0.20 0.50 ],[0.42 0.20 0.20 ]);
      | plot([0.20 0.10 0.30 0.20 ],[0.58 0.42 0.42 0.58 ],[0.10 0.30 ],[0.58 0.58 ]);
      | port_label('LConn',1,'D');
      | port_label('RConn',1,'S');
  QB_high : Subsystem  mask(PRISM-Hub switch cell){Ron=TB.B.Ron, Goff=TB.B.Goff, Vf=TB.B.Vf, Rd=TB.B.Rd, Goffd=TB.B.Goffd, Coss=TB.B.Coss_h}
      mask prompts: Ron "도통 저항 R_on [Ohm]"; Goff "차단 컨덕턴스 G_off [S]"; Vf "다이오드 순방향 전압 Vf [V]"; Rd "다이오드 도통 저항 R_d [Ohm]"; Goffd "다이오드 차단 컨덕턴스 [S]"; Coss "출력용량 C_oss [F]"
      mask help: 전력 반도체 스위치 셀 QB_H. 게이트 태그 gB_BH.
      settings: AttributesFormatString=gate: gB_BH
      mask Display:
      | plot([0.50 0.50 ],[0.95 0.65 ],[0.50 0.74 ],[0.65 0.35 ],[0.50 0.50 ],[0.35 0.05 ]);
      | plot([0.50 0.20 0.20 ],[0.80 0.80 0.58 ],[0.20 0.20 0.50 ],[0.42 0.20 0.20 ]);
      | plot([0.20 0.10 0.30 0.20 ],[0.58 0.42 0.42 0.58 ],[0.10 0.30 ],[0.58 0.58 ]);
      | port_label('LConn',1,'D');
      | port_label('RConn',1,'S');
  QB_low : Subsystem  mask(PRISM-Hub switch cell){Ron=TB.B.Ron, Goff=TB.B.Goff, Vf=TB.B.Vf, Rd=TB.B.Rd, Goffd=TB.B.Goffd, Coss=TB.B.Coss_h}
      mask prompts: Ron "도통 저항 R_on [Ohm]"; Goff "차단 컨덕턴스 G_off [S]"; Vf "다이오드 순방향 전압 Vf [V]"; Rd "다이오드 도통 저항 R_d [Ohm]"; Goffd "다이오드 차단 컨덕턴스 [S]"; Coss "출력용량 C_oss [F]"
      mask help: 전력 반도체 스위치 셀 QB_L. 게이트 태그 gB_BL.
      settings: AttributesFormatString=gate: gB_BL
      mask Display:
      | plot([0.50 0.50 ],[0.95 0.65 ],[0.50 0.74 ],[0.65 0.35 ],[0.50 0.50 ],[0.35 0.05 ]);
      | plot([0.50 0.20 0.20 ],[0.80 0.80 0.58 ],[0.20 0.20 0.50 ],[0.42 0.20 0.20 ]);
      | plot([0.20 0.10 0.30 0.20 ],[0.58 0.42 0.42 0.58 ],[0.10 0.30 ],[0.58 0.58 ]);
      | port_label('LConn',1,'D');
      | port_label('RConn',1,'S');
  V_nodeA : fl_lib/Electrical/Electrical Sensors/Voltage Sensor
  vA_node_PS2SL : nesl_utility/PS-Simulink Converter  PhysicalDomain=network_engine_domain  SubClassName=ps_output  LeftPortType=input  RightPortType=output  PseudoPeriodic=off  Frequencies=[]  VectorFormat=inherit  Unit=inherit  AffineConversion=off
  LINK_P : PMIOPort  Side=Left
  LINK_N : PMIOPort  Port=2  Side=Left
  A : PMIOPort  Port=3  Side=Right
  B : PMIOPort  Port=4  Side=Right
  tag scope: vA_node=global
  wires:
  vA_node_PS2SL/1 -> [vA_node]
  connections:
  QA_high/LConn1 -- LINK_P/RConn1 -- QB_high/LConn1
  QA_high/RConn1 -- A/RConn1 -- QA_low/LConn1 -- V_nodeA/LConn1
  QB_low/LConn1 -- QB_high/RConn1 -- B/RConn1
  QA_low/RConn1 -- QB_low/RConn1 -- LINK_N/RConn1 -- V_nodeA/RConn2
  V_nodeA/RConn1 -- vA_node_PS2SL/LConn1

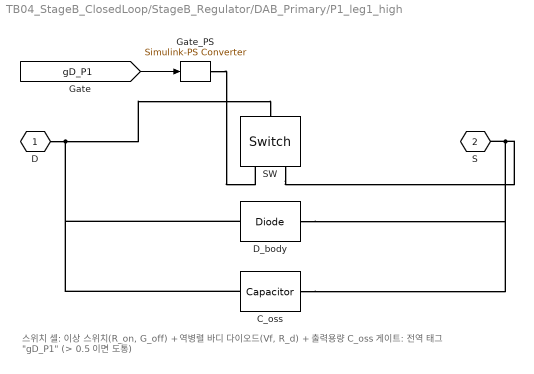
== system TB04_StageB_ClosedLoop/StageB_Regulator/DAB_Primary/P1_leg1_high ==
  note: 스위치 셀: 이상 스위치(R_on, G_off) + 역병렬 바디 다이오드(Vf, R_d) + 출력용량 C_oss
      | 게이트: 전역 태그 "gD_P1" (> 0.5 이면 도통)
  C_oss : fl_lib/Electrical/Electrical Elements/Capacitor  c=Coss F  r=1e-6 Ohm  g=0 1/Ohm  i_specify=off  i_priority=None  i=0 A  i_nominal_specify=off  i_nominal_value=1  i_nominal_unit=A  v_specify=off  v_priority=None  v=0 V  v_nominal_specify=off  v_nominal_value=1  v_nominal_unit=V  vc_specify=off  vc_priority=High  vc=0 V  vc_nominal_specify=off  vc_nominal_value=1  vc_nominal_unit=V
  D_body : fl_lib/Electrical/Electrical Elements/Diode  Vf=Vf V  Ron=Rd Ohm  Goff=Goffd 1/Ohm  i_specify=off  i_priority=None  i=0 A  i_nominal_specify=off  i_nominal_value=1  i_nominal_unit=A  v_specify=off  v_priority=None  v=0 V  v_nominal_specify=off  v_nominal_value=1  v_nominal_unit=V
  Gate_PS : nesl_utility/Simulink-PS Converter  PhysicalDomain=network_engine_domain  SubClassName=ps_input  LeftPortType=input  RightPortType=output  PseudoPeriodic=off  Frequencies=[]  NoiseDistribution=none  NoiseParameters=[]  Unit=1  AffineConversion=off  FilteringAndDerivatives=zero  SimscapeFilterOrder=1  InputFilterTimeConstant=0.001  UdotUserProvided=0
  SW : fl_lib/Electrical/Electrical Elements/Switch  R_closed=Ron Ohm  G_open=Goff 1/Ohm  Threshold=0.5  i_specify=off  i_priority=None  i=0 A  i_nominal_specify=off  i_nominal_value=1  i_nominal_unit=A  v_specify=off  v_priority=None  v=0 V  v_nominal_specify=off  v_nominal_value=1  v_nominal_unit=V
  D : PMIOPort  Side=Left
  S : PMIOPort  Port=2  Side=Right
  wires:
  [gD_P1] -> Gate_PS/1
  connections:
  Gate_PS/RConn1 -- SW/RConn1
  SW/LConn1 -- D/RConn1 -- D_body/RConn1 -- C_oss/LConn1
  SW/RConn2 -- D_body/LConn1 -- S/RConn1 -- C_oss/RConn1

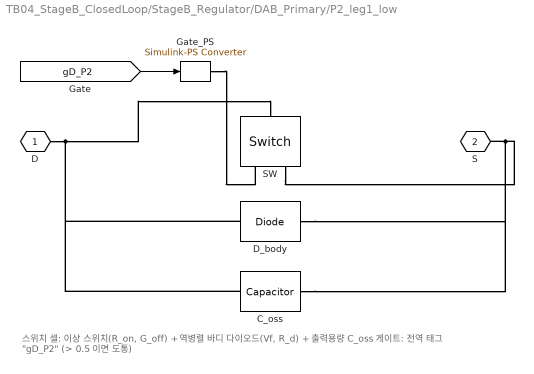
== system TB04_StageB_ClosedLoop/StageB_Regulator/DAB_Primary/P2_leg1_low ==
  note: 스위치 셀: 이상 스위치(R_on, G_off) + 역병렬 바디 다이오드(Vf, R_d) + 출력용량 C_oss
      | 게이트: 전역 태그 "gD_P2" (> 0.5 이면 도통)
  C_oss : fl_lib/Electrical/Electrical Elements/Capacitor  c=Coss F  r=1e-6 Ohm  g=0 1/Ohm  i_specify=off  i_priority=None  i=0 A  i_nominal_specify=off  i_nominal_value=1  i_nominal_unit=A  v_specify=off  v_priority=None  v=0 V  v_nominal_specify=off  v_nominal_value=1  v_nominal_unit=V  vc_specify=off  vc_priority=High  vc=0 V  vc_nominal_specify=off  vc_nominal_value=1  vc_nominal_unit=V
  D_body : fl_lib/Electrical/Electrical Elements/Diode  Vf=Vf V  Ron=Rd Ohm  Goff=Goffd 1/Ohm  i_specify=off  i_priority=None  i=0 A  i_nominal_specify=off  i_nominal_value=1  i_nominal_unit=A  v_specify=off  v_priority=None  v=0 V  v_nominal_specify=off  v_nominal_value=1  v_nominal_unit=V
  Gate_PS : nesl_utility/Simulink-PS Converter  PhysicalDomain=network_engine_domain  SubClassName=ps_input  LeftPortType=input  RightPortType=output  PseudoPeriodic=off  Frequencies=[]  NoiseDistribution=none  NoiseParameters=[]  Unit=1  AffineConversion=off  FilteringAndDerivatives=zero  SimscapeFilterOrder=1  InputFilterTimeConstant=0.001  UdotUserProvided=0
  SW : fl_lib/Electrical/Electrical Elements/Switch  R_closed=Ron Ohm  G_open=Goff 1/Ohm  Threshold=0.5  i_specify=off  i_priority=None  i=0 A  i_nominal_specify=off  i_nominal_value=1  i_nominal_unit=A  v_specify=off  v_priority=None  v=0 V  v_nominal_specify=off  v_nominal_value=1  v_nominal_unit=V
  D : PMIOPort  Side=Left
  S : PMIOPort  Port=2  Side=Right
  wires:
  [gD_P2] -> Gate_PS/1
  connections:
  Gate_PS/RConn1 -- SW/RConn1
  SW/LConn1 -- D/RConn1 -- D_body/RConn1 -- C_oss/LConn1
  SW/RConn2 -- D_body/LConn1 -- S/RConn1 -- C_oss/RConn1

== system TB04_StageB_ClosedLoop/StageB_Regulator/DAB_Primary/P3_leg2_high ==
  note: 스위치 셀: 이상 스위치(R_on, G_off) + 역병렬 바디 다이오드(Vf, R_d) + 출력용량 C_oss
      | 게이트: 전역 태그 "gD_P3" (> 0.5 이면 도통)
  C_oss : fl_lib/Electrical/Electrical Elements/Capacitor  c=Coss F  r=1e-6 Ohm  g=0 1/Ohm  i_specify=off  i_priority=None  i=0 A  i_nominal_specify=off  i_nominal_value=1  i_nominal_unit=A  v_specify=off  v_priority=None  v=0 V  v_nominal_specify=off  v_nominal_value=1  v_nominal_unit=V  vc_specify=off  vc_priority=High  vc=0 V  vc_nominal_specify=off  vc_nominal_value=1  vc_nominal_unit=V
  D_body : fl_lib/Electrical/Electrical Elements/Diode  Vf=Vf V  Ron=Rd Ohm  Goff=Goffd 1/Ohm  i_specify=off  i_priority=None  i=0 A  i_nominal_specify=off  i_nominal_value=1  i_nominal_unit=A  v_specify=off  v_priority=None  v=0 V  v_nominal_specify=off  v_nominal_value=1  v_nominal_unit=V
  Gate_PS : nesl_utility/Simulink-PS Converter  PhysicalDomain=network_engine_domain  SubClassName=ps_input  LeftPortType=input  RightPortType=output  PseudoPeriodic=off  Frequencies=[]  NoiseDistribution=none  NoiseParameters=[]  Unit=1  AffineConversion=off  FilteringAndDerivatives=zero  SimscapeFilterOrder=1  InputFilterTimeConstant=0.001  UdotUserProvided=0
  SW : fl_lib/Electrical/Electrical Elements/Switch  R_closed=Ron Ohm  G_open=Goff 1/Ohm  Threshold=0.5  i_specify=off  i_priority=None  i=0 A  i_nominal_specify=off  i_nominal_value=1  i_nominal_unit=A  v_specify=off  v_priority=None  v=0 V  v_nominal_specify=off  v_nominal_value=1  v_nominal_unit=V
  D : PMIOPort  Side=Left
  S : PMIOPort  Port=2  Side=Right
  wires:
  [gD_P3] -> Gate_PS/1
  connections:
  Gate_PS/RConn1 -- SW/RConn1
  SW/LConn1 -- D/RConn1 -- D_body/RConn1 -- C_oss/LConn1
  SW/RConn2 -- D_body/LConn1 -- S/RConn1 -- C_oss/RConn1

== system TB04_StageB_ClosedLoop/StageB_Regulator/DAB_Primary/P4_leg2_low ==
  note: 스위치 셀: 이상 스위치(R_on, G_off) + 역병렬 바디 다이오드(Vf, R_d) + 출력용량 C_oss
      | 게이트: 전역 태그 "gD_P4" (> 0.5 이면 도통)
  C_oss : fl_lib/Electrical/Electrical Elements/Capacitor  c=Coss F  r=1e-6 Ohm  g=0 1/Ohm  i_specify=off  i_priority=None  i=0 A  i_nominal_specify=off  i_nominal_value=1  i_nominal_unit=A  v_specify=off  v_priority=None  v=0 V  v_nominal_specify=off  v_nominal_value=1  v_nominal_unit=V  vc_specify=off  vc_priority=High  vc=0 V  vc_nominal_specify=off  vc_nominal_value=1  vc_nominal_unit=V
  D_body : fl_lib/Electrical/Electrical Elements/Diode  Vf=Vf V  Ron=Rd Ohm  Goff=Goffd 1/Ohm  i_specify=off  i_priority=None  i=0 A  i_nominal_specify=off  i_nominal_value=1  i_nominal_unit=A  v_specify=off  v_priority=None  v=0 V  v_nominal_specify=off  v_nominal_value=1  v_nominal_unit=V
  Gate_PS : nesl_utility/Simulink-PS Converter  PhysicalDomain=network_engine_domain  SubClassName=ps_input  LeftPortType=input  RightPortType=output  PseudoPeriodic=off  Frequencies=[]  NoiseDistribution=none  NoiseParameters=[]  Unit=1  AffineConversion=off  FilteringAndDerivatives=zero  SimscapeFilterOrder=1  InputFilterTimeConstant=0.001  UdotUserProvided=0
  SW : fl_lib/Electrical/Electrical Elements/Switch  R_closed=Ron Ohm  G_open=Goff 1/Ohm  Threshold=0.5  i_specify=off  i_priority=None  i=0 A  i_nominal_specify=off  i_nominal_value=1  i_nominal_unit=A  v_specify=off  v_priority=None  v=0 V  v_nominal_specify=off  v_nominal_value=1  v_nominal_unit=V
  D : PMIOPort  Side=Left
  S : PMIOPort  Port=2  Side=Right
  wires:
  [gD_P4] -> Gate_PS/1
  connections:
  Gate_PS/RConn1 -- SW/RConn1
  SW/LConn1 -- D/RConn1 -- D_body/RConn1 -- C_oss/LConn1
  SW/RConn2 -- D_body/LConn1 -- S/RConn1 -- C_oss/RConn1

== system TB04_StageB_ClosedLoop/StageB_Regulator/DAB_Secondary/S1_leg1_high ==
  note: 스위치 셀: 이상 스위치(R_on, G_off) + 역병렬 바디 다이오드(Vf, R_d) + 출력용량 C_oss
      | 게이트: 전역 태그 "gD_S1" (> 0.5 이면 도통)
  C_oss : fl_lib/Electrical/Electrical Elements/Capacitor  c=Coss F  r=1e-6 Ohm  g=0 1/Ohm  i_specify=off  i_priority=None  i=0 A  i_nominal_specify=off  i_nominal_value=1  i_nominal_unit=A  v_specify=off  v_priority=None  v=0 V  v_nominal_specify=off  v_nominal_value=1  v_nominal_unit=V  vc_specify=off  vc_priority=High  vc=0 V  vc_nominal_specify=off  vc_nominal_value=1  vc_nominal_unit=V
  D_body : fl_lib/Electrical/Electrical Elements/Diode  Vf=Vf V  Ron=Rd Ohm  Goff=Goffd 1/Ohm  i_specify=off  i_priority=None  i=0 A  i_nominal_specify=off  i_nominal_value=1  i_nominal_unit=A  v_specify=off  v_priority=None  v=0 V  v_nominal_specify=off  v_nominal_value=1  v_nominal_unit=V
  Gate_PS : nesl_utility/Simulink-PS Converter  PhysicalDomain=network_engine_domain  SubClassName=ps_input  LeftPortType=input  RightPortType=output  PseudoPeriodic=off  Frequencies=[]  NoiseDistribution=none  NoiseParameters=[]  Unit=1  AffineConversion=off  FilteringAndDerivatives=zero  SimscapeFilterOrder=1  InputFilterTimeConstant=0.001  UdotUserProvided=0
  SW : fl_lib/Electrical/Electrical Elements/Switch  R_closed=Ron Ohm  G_open=Goff 1/Ohm  Threshold=0.5  i_specify=off  i_priority=None  i=0 A  i_nominal_specify=off  i_nominal_value=1  i_nominal_unit=A  v_specify=off  v_priority=None  v=0 V  v_nominal_specify=off  v_nominal_value=1  v_nominal_unit=V
  D : PMIOPort  Side=Left
  S : PMIOPort  Port=2  Side=Right
  wires:
  [gD_S1] -> Gate_PS/1
  connections:
  Gate_PS/RConn1 -- SW/RConn1
  SW/LConn1 -- D/RConn1 -- D_body/RConn1 -- C_oss/LConn1
  SW/RConn2 -- D_body/LConn1 -- S/RConn1 -- C_oss/RConn1

== system TB04_StageB_ClosedLoop/StageB_Regulator/DAB_Secondary/S2_leg1_low ==
  note: 스위치 셀: 이상 스위치(R_on, G_off) + 역병렬 바디 다이오드(Vf, R_d) + 출력용량 C_oss
      | 게이트: 전역 태그 "gD_S2" (> 0.5 이면 도통)
  C_oss : fl_lib/Electrical/Electrical Elements/Capacitor  c=Coss F  r=1e-6 Ohm  g=0 1/Ohm  i_specify=off  i_priority=None  i=0 A  i_nominal_specify=off  i_nominal_value=1  i_nominal_unit=A  v_specify=off  v_priority=None  v=0 V  v_nominal_specify=off  v_nominal_value=1  v_nominal_unit=V  vc_specify=off  vc_priority=High  vc=0 V  vc_nominal_specify=off  vc_nominal_value=1  vc_nominal_unit=V
  D_body : fl_lib/Electrical/Electrical Elements/Diode  Vf=Vf V  Ron=Rd Ohm  Goff=Goffd 1/Ohm  i_specify=off  i_priority=None  i=0 A  i_nominal_specify=off  i_nominal_value=1  i_nominal_unit=A  v_specify=off  v_priority=None  v=0 V  v_nominal_specify=off  v_nominal_value=1  v_nominal_unit=V
  Gate_PS : nesl_utility/Simulink-PS Converter  PhysicalDomain=network_engine_domain  SubClassName=ps_input  LeftPortType=input  RightPortType=output  PseudoPeriodic=off  Frequencies=[]  NoiseDistribution=none  NoiseParameters=[]  Unit=1  AffineConversion=off  FilteringAndDerivatives=zero  SimscapeFilterOrder=1  InputFilterTimeConstant=0.001  UdotUserProvided=0
  SW : fl_lib/Electrical/Electrical Elements/Switch  R_closed=Ron Ohm  G_open=Goff 1/Ohm  Threshold=0.5  i_specify=off  i_priority=None  i=0 A  i_nominal_specify=off  i_nominal_value=1  i_nominal_unit=A  v_specify=off  v_priority=None  v=0 V  v_nominal_specify=off  v_nominal_value=1  v_nominal_unit=V
  D : PMIOPort  Side=Left
  S : PMIOPort  Port=2  Side=Right
  wires:
  [gD_S2] -> Gate_PS/1
  connections:
  Gate_PS/RConn1 -- SW/RConn1
  SW/LConn1 -- D/RConn1 -- D_body/RConn1 -- C_oss/LConn1
  SW/RConn2 -- D_body/LConn1 -- S/RConn1 -- C_oss/RConn1

== system TB04_StageB_ClosedLoop/StageB_Regulator/DAB_Secondary/S3_leg2_high ==
  note: 스위치 셀: 이상 스위치(R_on, G_off) + 역병렬 바디 다이오드(Vf, R_d) + 출력용량 C_oss
      | 게이트: 전역 태그 "gD_S3" (> 0.5 이면 도통)
  C_oss : fl_lib/Electrical/Electrical Elements/Capacitor  c=Coss F  r=1e-6 Ohm  g=0 1/Ohm  i_specify=off  i_priority=None  i=0 A  i_nominal_specify=off  i_nominal_value=1  i_nominal_unit=A  v_specify=off  v_priority=None  v=0 V  v_nominal_specify=off  v_nominal_value=1  v_nominal_unit=V  vc_specify=off  vc_priority=High  vc=0 V  vc_nominal_specify=off  vc_nominal_value=1  vc_nominal_unit=V
  D_body : fl_lib/Electrical/Electrical Elements/Diode  Vf=Vf V  Ron=Rd Ohm  Goff=Goffd 1/Ohm  i_specify=off  i_priority=None  i=0 A  i_nominal_specify=off  i_nominal_value=1  i_nominal_unit=A  v_specify=off  v_priority=None  v=0 V  v_nominal_specify=off  v_nominal_value=1  v_nominal_unit=V
  Gate_PS : nesl_utility/Simulink-PS Converter  PhysicalDomain=network_engine_domain  SubClassName=ps_input  LeftPortType=input  RightPortType=output  PseudoPeriodic=off  Frequencies=[]  NoiseDistribution=none  NoiseParameters=[]  Unit=1  AffineConversion=off  FilteringAndDerivatives=zero  SimscapeFilterOrder=1  InputFilterTimeConstant=0.001  UdotUserProvided=0
  SW : fl_lib/Electrical/Electrical Elements/Switch  R_closed=Ron Ohm  G_open=Goff 1/Ohm  Threshold=0.5  i_specify=off  i_priority=None  i=0 A  i_nominal_specify=off  i_nominal_value=1  i_nominal_unit=A  v_specify=off  v_priority=None  v=0 V  v_nominal_specify=off  v_nominal_value=1  v_nominal_unit=V
  D : PMIOPort  Side=Left
  S : PMIOPort  Port=2  Side=Right
  wires:
  [gD_S3] -> Gate_PS/1
  connections:
  Gate_PS/RConn1 -- SW/RConn1
  SW/LConn1 -- D/RConn1 -- D_body/RConn1 -- C_oss/LConn1
  SW/RConn2 -- D_body/LConn1 -- S/RConn1 -- C_oss/RConn1

== system TB04_StageB_ClosedLoop/StageB_Regulator/DAB_Secondary/S4_leg2_low ==
  note: 스위치 셀: 이상 스위치(R_on, G_off) + 역병렬 바디 다이오드(Vf, R_d) + 출력용량 C_oss
      | 게이트: 전역 태그 "gD_S4" (> 0.5 이면 도통)
  C_oss : fl_lib/Electrical/Electrical Elements/Capacitor  c=Coss F  r=1e-6 Ohm  g=0 1/Ohm  i_specify=off  i_priority=None  i=0 A  i_nominal_specify=off  i_nominal_value=1  i_nominal_unit=A  v_specify=off  v_priority=None  v=0 V  v_nominal_specify=off  v_nominal_value=1  v_nominal_unit=V  vc_specify=off  vc_priority=High  vc=0 V  vc_nominal_specify=off  vc_nominal_value=1  vc_nominal_unit=V
  D_body : fl_lib/Electrical/Electrical Elements/Diode  Vf=Vf V  Ron=Rd Ohm  Goff=Goffd 1/Ohm  i_specify=off  i_priority=None  i=0 A  i_nominal_specify=off  i_nominal_value=1  i_nominal_unit=A  v_specify=off  v_priority=None  v=0 V  v_nominal_specify=off  v_nominal_value=1  v_nominal_unit=V
  Gate_PS : nesl_utility/Simulink-PS Converter  PhysicalDomain=network_engine_domain  SubClassName=ps_input  LeftPortType=input  RightPortType=output  PseudoPeriodic=off  Frequencies=[]  NoiseDistribution=none  NoiseParameters=[]  Unit=1  AffineConversion=off  FilteringAndDerivatives=zero  SimscapeFilterOrder=1  InputFilterTimeConstant=0.001  UdotUserProvided=0
  SW : fl_lib/Electrical/Electrical Elements/Switch  R_closed=Ron Ohm  G_open=Goff 1/Ohm  Threshold=0.5  i_specify=off  i_priority=None  i=0 A  i_nominal_specify=off  i_nominal_value=1  i_nominal_unit=A  v_specify=off  v_priority=None  v=0 V  v_nominal_specify=off  v_nominal_value=1  v_nominal_unit=V
  D : PMIOPort  Side=Left
  S : PMIOPort  Port=2  Side=Right
  wires:
  [gD_S4] -> Gate_PS/1
  connections:
  Gate_PS/RConn1 -- SW/RConn1
  SW/LConn1 -- D/RConn1 -- D_body/RConn1 -- C_oss/LConn1
  SW/RConn2 -- D_body/LConn1 -- S/RConn1 -- C_oss/RConn1

== system TB04_StageB_ClosedLoop/StageB_Regulator/HBridge/QA_high ==
  note: 스위치 셀: 이상 스위치(R_on, G_off) + 역병렬 바디 다이오드(Vf, R_d) + 출력용량 C_oss
      | 게이트: 전역 태그 "gB_AH" (> 0.5 이면 도통)
  C_oss : fl_lib/Electrical/Electrical Elements/Capacitor  c=Coss F  r=1e-6 Ohm  g=0 1/Ohm  i_specify=off  i_priority=None  i=0 A  i_nominal_specify=off  i_nominal_value=1  i_nominal_unit=A  v_specify=off  v_priority=None  v=0 V  v_nominal_specify=off  v_nominal_value=1  v_nominal_unit=V  vc_specify=off  vc_priority=High  vc=0 V  vc_nominal_specify=off  vc_nominal_value=1  vc_nominal_unit=V
  D_body : fl_lib/Electrical/Electrical Elements/Diode  Vf=Vf V  Ron=Rd Ohm  Goff=Goffd 1/Ohm  i_specify=off  i_priority=None  i=0 A  i_nominal_specify=off  i_nominal_value=1  i_nominal_unit=A  v_specify=off  v_priority=None  v=0 V  v_nominal_specify=off  v_nominal_value=1  v_nominal_unit=V
  Gate_PS : nesl_utility/Simulink-PS Converter  PhysicalDomain=network_engine_domain  SubClassName=ps_input  LeftPortType=input  RightPortType=output  PseudoPeriodic=off  Frequencies=[]  NoiseDistribution=none  NoiseParameters=[]  Unit=1  AffineConversion=off  FilteringAndDerivatives=zero  SimscapeFilterOrder=1  InputFilterTimeConstant=0.001  UdotUserProvided=0
  SW : fl_lib/Electrical/Electrical Elements/Switch  R_closed=Ron Ohm  G_open=Goff 1/Ohm  Threshold=0.5  i_specify=off  i_priority=None  i=0 A  i_nominal_specify=off  i_nominal_value=1  i_nominal_unit=A  v_specify=off  v_priority=None  v=0 V  v_nominal_specify=off  v_nominal_value=1  v_nominal_unit=V
  D : PMIOPort  Side=Left
  S : PMIOPort  Port=2  Side=Right
  wires:
  [gB_AH] -> Gate_PS/1
  connections:
  Gate_PS/RConn1 -- SW/RConn1
  SW/LConn1 -- D/RConn1 -- D_body/RConn1 -- C_oss/LConn1
  SW/RConn2 -- D_body/LConn1 -- S/RConn1 -- C_oss/RConn1

== system TB04_StageB_ClosedLoop/StageB_Regulator/HBridge/QA_low ==
  note: 스위치 셀: 이상 스위치(R_on, G_off) + 역병렬 바디 다이오드(Vf, R_d) + 출력용량 C_oss
      | 게이트: 전역 태그 "gB_AL" (> 0.5 이면 도통)
  C_oss : fl_lib/Electrical/Electrical Elements/Capacitor  c=Coss F  r=1e-6 Ohm  g=0 1/Ohm  i_specify=off  i_priority=None  i=0 A  i_nominal_specify=off  i_nominal_value=1  i_nominal_unit=A  v_specify=off  v_priority=None  v=0 V  v_nominal_specify=off  v_nominal_value=1  v_nominal_unit=V  vc_specify=off  vc_priority=High  vc=0 V  vc_nominal_specify=off  vc_nominal_value=1  vc_nominal_unit=V
  D_body : fl_lib/Electrical/Electrical Elements/Diode  Vf=Vf V  Ron=Rd Ohm  Goff=Goffd 1/Ohm  i_specify=off  i_priority=None  i=0 A  i_nominal_specify=off  i_nominal_value=1  i_nominal_unit=A  v_specify=off  v_priority=None  v=0 V  v_nominal_specify=off  v_nominal_value=1  v_nominal_unit=V
  Gate_PS : nesl_utility/Simulink-PS Converter  PhysicalDomain=network_engine_domain  SubClassName=ps_input  LeftPortType=input  RightPortType=output  PseudoPeriodic=off  Frequencies=[]  NoiseDistribution=none  NoiseParameters=[]  Unit=1  AffineConversion=off  FilteringAndDerivatives=zero  SimscapeFilterOrder=1  InputFilterTimeConstant=0.001  UdotUserProvided=0
  SW : fl_lib/Electrical/Electrical Elements/Switch  R_closed=Ron Ohm  G_open=Goff 1/Ohm  Threshold=0.5  i_specify=off  i_priority=None  i=0 A  i_nominal_specify=off  i_nominal_value=1  i_nominal_unit=A  v_specify=off  v_priority=None  v=0 V  v_nominal_specify=off  v_nominal_value=1  v_nominal_unit=V
  D : PMIOPort  Side=Left
  S : PMIOPort  Port=2  Side=Right
  wires:
  [gB_AL] -> Gate_PS/1
  connections:
  Gate_PS/RConn1 -- SW/RConn1
  SW/LConn1 -- D/RConn1 -- D_body/RConn1 -- C_oss/LConn1
  SW/RConn2 -- D_body/LConn1 -- S/RConn1 -- C_oss/RConn1

== system TB04_StageB_ClosedLoop/StageB_Regulator/HBridge/QB_high ==
  note: 스위치 셀: 이상 스위치(R_on, G_off) + 역병렬 바디 다이오드(Vf, R_d) + 출력용량 C_oss
      | 게이트: 전역 태그 "gB_BH" (> 0.5 이면 도통)
  C_oss : fl_lib/Electrical/Electrical Elements/Capacitor  c=Coss F  r=1e-6 Ohm  g=0 1/Ohm  i_specify=off  i_priority=None  i=0 A  i_nominal_specify=off  i_nominal_value=1  i_nominal_unit=A  v_specify=off  v_priority=None  v=0 V  v_nominal_specify=off  v_nominal_value=1  v_nominal_unit=V  vc_specify=off  vc_priority=High  vc=0 V  vc_nominal_specify=off  vc_nominal_value=1  vc_nominal_unit=V
  D_body : fl_lib/Electrical/Electrical Elements/Diode  Vf=Vf V  Ron=Rd Ohm  Goff=Goffd 1/Ohm  i_specify=off  i_priority=None  i=0 A  i_nominal_specify=off  i_nominal_value=1  i_nominal_unit=A  v_specify=off  v_priority=None  v=0 V  v_nominal_specify=off  v_nominal_value=1  v_nominal_unit=V
  Gate_PS : nesl_utility/Simulink-PS Converter  PhysicalDomain=network_engine_domain  SubClassName=ps_input  LeftPortType=input  RightPortType=output  PseudoPeriodic=off  Frequencies=[]  NoiseDistribution=none  NoiseParameters=[]  Unit=1  AffineConversion=off  FilteringAndDerivatives=zero  SimscapeFilterOrder=1  InputFilterTimeConstant=0.001  UdotUserProvided=0
  SW : fl_lib/Electrical/Electrical Elements/Switch  R_closed=Ron Ohm  G_open=Goff 1/Ohm  Threshold=0.5  i_specify=off  i_priority=None  i=0 A  i_nominal_specify=off  i_nominal_value=1  i_nominal_unit=A  v_specify=off  v_priority=None  v=0 V  v_nominal_specify=off  v_nominal_value=1  v_nominal_unit=V
  D : PMIOPort  Side=Left
  S : PMIOPort  Port=2  Side=Right
  wires:
  [gB_BH] -> Gate_PS/1
  connections:
  Gate_PS/RConn1 -- SW/RConn1
  SW/LConn1 -- D/RConn1 -- D_body/RConn1 -- C_oss/LConn1
  SW/RConn2 -- D_body/LConn1 -- S/RConn1 -- C_oss/RConn1
